simulink model "Mega_Demo_All"  (R2013a)
settings: Solver=FixedStepDiscrete  SolverMode=SingleTasking  StartTime=0.0  StopTime=inf  FixedStep=.1  RelTol=1e-3
libraries: arduinolib x5
settings Model: SimulationMode=external  ExtModeTrigDuration=2  Creator=Alec  LastModifiedBy=hurstj
settings OptimizationCC: ExpressionDepthLimit=2147483647  OptimizeModelRefInitCode=on  LifeSpan=1
settings DebuggingCC: SolverPrmCheckMsg=none  StrictBusMsg=Warning
settings HardwareCC: ProdBitPerInt=16  ProdBitPerPointer=8  ProdIntDivRoundTo=Zero  ProdEndianess=LittleEndian  ProdWordSize=8  ProdHWDeviceType=Atmel->AVR
settings RTWCC: SystemTargetFile=realtime.tlc  GenerateMakefile=off  TemplateMakefile=realtime.tmf  Description=Real-Time Toolbox  RTWVerbose=off  ProcessScript=realtime_make_rtw_hook
settings CodeAppCC: CustomSymbolStrType=$N$R$M  InternalIdentifier=Classic
settings STFCustomTargetCC: TargetLibSuffix=.a  GenerateSampleERTMain=on  ERTCustomFileBanners=on  SupportNonInlinedSFcns=off  SupportVariableSizeSignals=on  MATLABClassNameForMDSCustomization=Simulink.SoftwareTarget.ERTCustomization  SystemTargetFile=realtime.tlc
settings ERTTargetCC: ParMdlRefBuildCompliant=off  CompOptLevelCompliant=off  ConcurrentExecutionCompliant=off  CombineOutputUpdateFcns=off  ERTFirstTimeCompliant=off  SupportContinuousTime=on  SupportVariableSizeSignals=on  ModelStepFunctionPrototypeControlCompliant=off  CPPClassGenCompliant=off  ExtMode=on  ExtModeTransport=3  ExtModeMexFile=ext_serial_win32_comm  ExtModeMexArgs=0 90 115200  ERTSrcFileBannerTemplate=realtime_code_template.cgt  ERTHdrFileBannerTemplate=realtime_code_template.cgt  ERTDataSrcFileTemplate=realtime_code_template.cgt  ERTDataHdrFileTemplate=realtime_code_template.cgt  ERTCustomFileTemplate=realtime_file_process.tlc

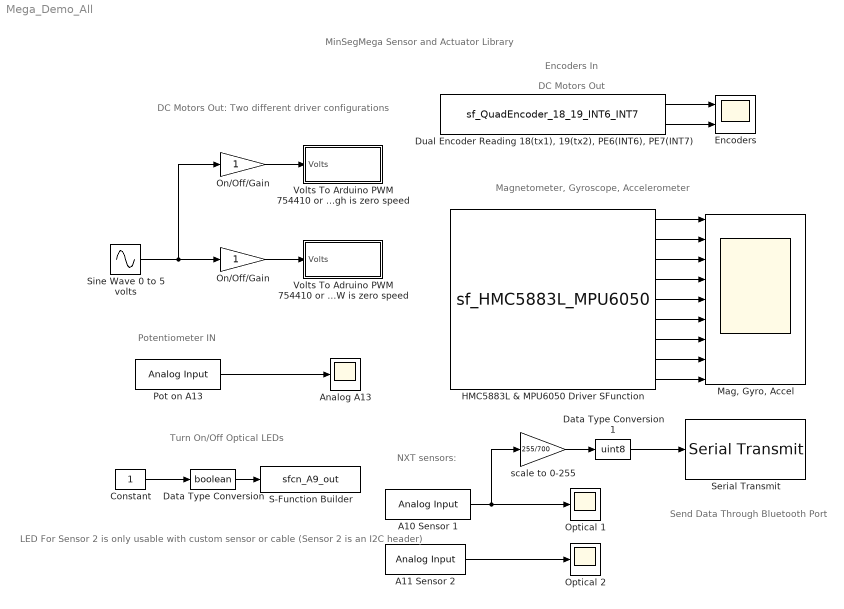
== system Mega_Demo_All ==
  note: MinSegMega Sensor and Actuator Library
  note: LED For Sensor 2 is only
      | usable with custom sensor
      | or cable (Sensor 2 is an I2C header)
  note: Turn On/Off Optical LEDs
  note: Send Data Through
      | Bluetooth Port
  note: Potentiometer IN
  note: DC Motors Out:
      | Two different driver configurations
  note: DC Motors Out
  note: Encoders In
  note: NXT sensors:
  note: Magnetometer, Gyroscope, Accelerometer
  A10 Sensor 1 : arduinolib/Analog Input  pinNumber=10  sampleTime=-1
  A11 Sensor 2 : arduinolib/Analog Input  pinNumber=11  sampleTime=-1
  Analog A13 : Scope
      settings: TimeRange=30  YMin=275  YMax=600  SaveName=ScopeData6
  Constant : Constant  SampleTime=-1
  Data Type Conversion : DataTypeConversion  OutDataTypeStr=boolean
  Data Type Conversion1 : DataTypeConversion  OutDataTypeStr=uint8
  "Dual Encoder Reading 18(tx1), 19(tx2), PE6(INT6), PE7(INT7) " : S-Function  InitFcn=try, set_param(gcb,'FunctionName','sf_QuadEncoder_18_19_INT6_INT7'), end  FunctionName=sf_QuadEncoder_18_19_INT6_INT7  Parameters=uint8([0 1]),uint8([18 6]),uint8([19 7])  SFunctionModules=sf_QuadEncoder_18_19_INT6_INT7_wrapper  EnableBusSupport=off  mask(S-Function Builder){}
      mask init:
      | val = [[.9  0.75 0.75 1 1 .9 .9 1]',[1 1 0.75 0.75 .9 .9 1 .9]'];try , sys = get_param(gcb,'SfunBuilderFcnName');if isempty(sys), sys = get_param(gcb,'FunctionName'); end,catch, sys = get_param(gcb,'FunctionName'); end
      settings: CopyFcn=set_param(gcbh,'LinkStatus','none')  PreSaveFcn=try, set_param(gcb,'FunctionName','sf_QuadEncoder_18_19_INT6_INT7'), end  OpenFcn=sfunctionwizard(gcbh)
      mask Display: plot(val(:,1),val(:,2)),disp(sys), port_label('output',1,'pos1'), port_label('output',2,'pos2')
  Encoders : Scope  NumInputPorts=2
      settings: TimeRange=30  YMin=-1500~0  YMax=750~1000
  HMC5883L & MPU6050 Driver SFunction : S-Function  InitFcn=try, set_param(gcb,'FunctionName','sf_HMC5883L_MPU6050'), end  FunctionName=sf_HMC5883L_MPU6050  SFunctionModules=sf_HMC5883L_MPU6050_wrapper  EnableBusSupport=off  mask(S-Function Builder){}
      mask help: Simulink:masks:SFunctionBuilder_MD
      mask init: same as Mega_Demo_All/Dual Encoder Reading 18(tx1), 19(tx2), PE6(INT6), PE7(INT7) 
      settings: CopyFcn=set_param(gcbh,'LinkStatus','none')  PreSaveFcn=try, set_param(gcb,'FunctionName','sf_HMC5883L_MPU6050'), end  OpenFcn=sfunctionwizard(gcbh)
      mask Display:
      | plot(val(:,1),val(:,2))
      | disp(sys)
      | port_label('output',1,'x_mag')
      | port_label('output',2,'y_mag')
      | port_label('output',3,'z_mag')
      | port_label('output',4,'x_vel')
      | port_label('output',5,'y_vel')
      | port_label('output',6,'z_vel')
      | port_label('output',7,'x_acc')
      | port_label('output',8,'y_acc')
      | port_label('output',9,'z_acc')
  "Mag, Gyro, Accel" : Scope  NumInputPorts=9
      settings: TimeRange=10  YMin=-225~-450~-1~-700~-400~-30000~-1000~-2500~15500  YMax=-100~-275~0~300~700~40000~4000~1000~18500
  On/Off/Gain : Gain  OutDataTypeStr=int16
  "On/Off/Gain " : Gain  OutDataTypeStr=int16
  Optical 1 : Scope
      settings: TimeRange=30  YMin=300  YMax=1100  SaveName=ScopeData4
  Optical 2 : Scope
      settings: TimeRange=30  YMin=100  YMax=1100  SaveName=ScopeData3
  Pot on A13 : arduinolib/Analog Input  pinNumber=13  sampleTime=-1
  S-Function Builder : S-Function  InitFcn=try, set_param(gcb,'FunctionName','sfcn_A9_out'), end  FunctionName=sfcn_A9_out  Parameters=uint8(9)  SFunctionModules=sfcn_A9_out_wrapper  EnableBusSupport=off  mask(S-Function Builder){}
      mask init: same as Mega_Demo_All/Dual Encoder Reading 18(tx1), 19(tx2), PE6(INT6), PE7(INT7) 
      settings: CopyFcn=set_param(gcbh,'LinkStatus','none')  PreSaveFcn=try, set_param(gcb,'FunctionName','sfcn_A9_out'), end  OpenFcn=sfunctionwizard(gcbh)
      mask Display: plot(val(:,1),val(:,2)),disp(sys), port_label('input',1,'in')
  Serial Transmit : arduinolib/Serial Transmit  portNumber=3
  Sine Wave 0 to 5 volts : Sin  SineType=Sample based  Amplitude=5  Frequency=50*2*pi  Samples=30  SampleTime=.1
  Volts To Adruino PWM 754410 or DRV8833 PWM LOW is zero speed : Subsystem
  Volts To Arduino PWM 754410 or DRV8833 PWM High is zero speed : Subsystem
  scale to 0-255 : Gain  Gain=255/700  OutDataTypeStr=int16
  wires:
  On/Off/Gain/1 -> Volts To Arduino PWM 754410 or DRV8833 PWM High is zero speed/1(Volts)
  Sine Wave 0 to 5 volts/1 -> "On/Off/Gain "/1, On/Off/Gain/1
  "On/Off/Gain "/1 -> Volts To Adruino PWM 754410 or DRV8833 PWM LOW is zero speed/1(Volts)
  "Dual Encoder Reading 18(tx1), 19(tx2), PE6(INT6), PE7(INT7) "/1 -> Encoders/1
  "Dual Encoder Reading 18(tx1), 19(tx2), PE6(INT6), PE7(INT7) "/2 -> Encoders/2
  A10 Sensor 1/1 -> scale to 0-255/1, Optical 1/1
  Constant/1 -> Data Type Conversion/1
  HMC5883L & MPU6050 Driver SFunction/1 -> "Mag, Gyro, Accel"/1
  HMC5883L & MPU6050 Driver SFunction/2 -> "Mag, Gyro, Accel"/2
  HMC5883L & MPU6050 Driver SFunction/3 -> "Mag, Gyro, Accel"/3
  HMC5883L & MPU6050 Driver SFunction/4 -> "Mag, Gyro, Accel"/4
  HMC5883L & MPU6050 Driver SFunction/5 -> "Mag, Gyro, Accel"/5
  HMC5883L & MPU6050 Driver SFunction/6 -> "Mag, Gyro, Accel"/6
  HMC5883L & MPU6050 Driver SFunction/7 -> "Mag, Gyro, Accel"/7
  HMC5883L & MPU6050 Driver SFunction/8 -> "Mag, Gyro, Accel"/8
  HMC5883L & MPU6050 Driver SFunction/9 -> "Mag, Gyro, Accel"/9
  scale to 0-255/1 -> Data Type Conversion1/1
  Data Type Conversion1/1 -> Serial Transmit/1
  A11 Sensor 2/1 -> Optical 2/1
  Pot on A13/1 -> Analog A13/1
  Data Type Conversion/1 -> S-Function Builder/1

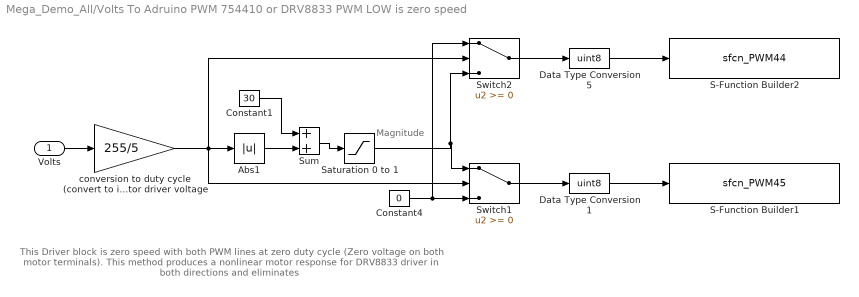
== system Mega_Demo_All/Volts To Adruino PWM 754410 or DRV8833 PWM LOW is zero speed ==
  note: Magnitude
  note: This Driver block is zero speed with both PWM lines at zero duty cycle
      |  (Zero voltage on both motor terminals).
      | This method produces a nonlinear motor response for DRV8833 driver
      |  in both directions and eliminates
  Volts : Inport
  Abs1 : Abs
  Constant1 : Constant  Value=30
  Constant4 : Constant  Value=0
  Data Type Conversion1 : DataTypeConversion  OutDataTypeStr=uint8
  Data Type Conversion5 : DataTypeConversion  OutDataTypeStr=uint8
  S-Function Builder1 : S-Function  InitFcn=try, set_param(gcb,'FunctionName','sfcn_PWM45'), end  FunctionName=sfcn_PWM45  Parameters=uint8(45)  SFunctionModules=sfcn_PWM45_wrapper  EnableBusSupport=off  mask(S-Function Builder){}
      mask init: same as Mega_Demo_All/Dual Encoder Reading 18(tx1), 19(tx2), PE6(INT6), PE7(INT7) 
      settings: CopyFcn=set_param(gcbh,'LinkStatus','none')  PreSaveFcn=try, set_param(gcb,'FunctionName','sfcn_PWM45'), end  OpenFcn=sfunctionwizard(gcbh)
      mask Display: plot(val(:,1),val(:,2)),disp(sys), port_label('input',1,'in')
  S-Function Builder2 : S-Function  InitFcn=try, set_param(gcb,'FunctionName','sfcn_PWM44'), end  FunctionName=sfcn_PWM44  Parameters=uint8(44)  SFunctionModules=sfcn_PWM44_wrapper  EnableBusSupport=off  mask(S-Function Builder){}
      mask init: same as Mega_Demo_All/Dual Encoder Reading 18(tx1), 19(tx2), PE6(INT6), PE7(INT7) 
      settings: CopyFcn=set_param(gcbh,'LinkStatus','none')  PreSaveFcn=try, set_param(gcb,'FunctionName','sfcn_PWM44'), end  OpenFcn=sfunctionwizard(gcbh)
      mask Display: plot(val(:,1),val(:,2)),disp(sys), port_label('input',1,'in')
  Saturation 0 to 1 : Saturate  UpperLimit=255  LowerLimit=0
  Sum : Sum
  Switch1 : Switch
  Switch2 : Switch
  conversion to duty cycle (convert to int) denominator is motor driver voltage : Gain  Gain=255/5  OutDataTypeStr=int16
  wires:
  Constant1/1 -> Sum/1
  Sum/1 -> Saturation 0 to 1/1
  Abs1/1 -> Sum/2
  Data Type Conversion1/1 -> S-Function Builder1/1
  Data Type Conversion5/1 -> S-Function Builder2/1
  Switch1/1 -> Data Type Conversion1/1
  Switch2/1 -> Data Type Conversion5/1
  Saturation 0 to 1/1 -> Switch1/1, Switch2/3
  Constant4/1 -> Switch1/3, Switch2/1
  conversion to duty cycle (convert to int) denominator is motor driver voltage/1 -> Switch2/2, Abs1/1, Switch1/2
  Volts/1 -> conversion to duty cycle (convert to int) denominator is motor driver voltage/1

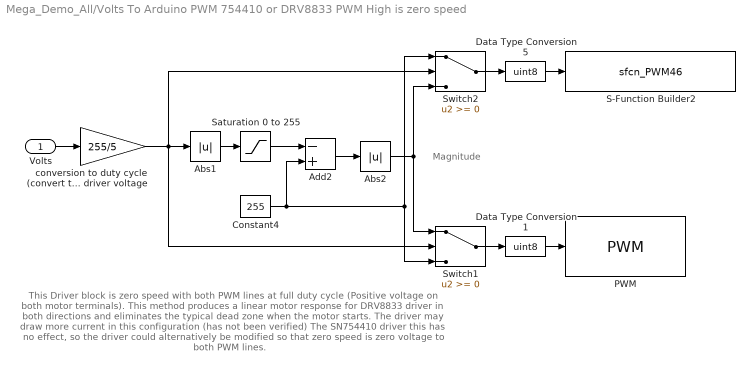
== system Mega_Demo_All/Volts To Arduino PWM 754410 or DRV8833 PWM High is zero speed ==
  note: This Driver block is zero speed with both PWM lines at full duty cycle
      |  (Positive voltage on both motor terminals).
      | This method produces a linear motor response for DRV8833 driver
      |  in both directions and eliminates
      | the typical dead zone when the motor starts.
      | The driver may draw more current in this configuration (has not been verified)
      |
      | The SN754410 driver this has no effect, so the driver could alternatively
      | be modified so that zero speed is zero voltage to both PWM lines.
  note: Magnitude
  Volts : Inport
  Abs1 : Abs
  Abs2 : Abs
  Add2 : Sum  Inputs=-+
  Constant4 : Constant  Value=255
  Data Type Conversion1 : DataTypeConversion  OutDataTypeStr=uint8
  Data Type Conversion5 : DataTypeConversion  OutDataTypeStr=uint8
  PWM : arduinolib/PWM  pinNumber=2
  S-Function Builder2 : S-Function  InitFcn=try, set_param(gcb,'FunctionName','sfcn_PWM46'), end  FunctionName=sfcn_PWM46  Parameters=uint8(46)  SFunctionModules=sfcn_PWM46_wrapper  EnableBusSupport=off  mask(S-Function Builder){}
      mask init: same as Mega_Demo_All/Dual Encoder Reading 18(tx1), 19(tx2), PE6(INT6), PE7(INT7) 
      settings: CopyFcn=set_param(gcbh,'LinkStatus','none')  PreSaveFcn=try, set_param(gcb,'FunctionName','sfcn_PWM46'), end  OpenFcn=sfunctionwizard(gcbh)
      mask Display: plot(val(:,1),val(:,2)),disp(sys), port_label('input',1,'in')
  Saturation 0 to 255 : Saturate  UpperLimit=255  LowerLimit=0
  Switch1 : Switch
  Switch2 : Switch
  conversion to duty cycle (convert to int) denominator is motor driver voltage : Gain  Gain=255/5  OutDataTypeStr=int16
  wires:
  Volts/1 -> conversion to duty cycle (convert to int) denominator is motor driver voltage/1
  conversion to duty cycle (convert to int) denominator is motor driver voltage/1 -> Abs1/1, Switch2/2, Switch1/2
  Saturation 0 to 255/1 -> Add2/1
  Abs1/1 -> Saturation 0 to 255/1
  Constant4/1 -> Switch1/3, Switch2/1, Add2/2
  Add2/1 -> Abs2/1
  Abs2/1 -> Switch2/3, Switch1/1
  Switch2/1 -> Data Type Conversion5/1
  Switch1/1 -> Data Type Conversion1/1
  Data Type Conversion5/1 -> S-Function Builder2/1
  Data Type Conversion1/1 -> PWM/1
